simulink model "Controller_torque_cbf"  (R2026b)
settings: Solver=ode4  StopTime=Inf  FixedStep=1e-3
values from neighbouring files (symbols this model uses):
  Dn = 20 * ones(7,1)    [init_torque_cbf.m]
  H_0_cy = H_0_pr * H_pr_cy    [init_torque_cbf.m]
  H_home = getTransform(Franka_robot, q_home, 'panda_link8', 'panda_link0')    [init_torque_cbf.m]
  Kn = 0 * ones(7,1)    [init_torque_cbf.m]
  q_home = q_init    [init_torque_cbf.m]
  q_init = [0 0  0  -(2/4)*pi  0  pi/2  -pi/4]'    [init_torque_cbf.m]
undefined symbols (not defined in the file or in its folder): cbf_torque_params, DiscIntNeverNeededParam, Fext_mag, T_final, X, Y, Z
libraries: sm_lib x162, nesl_utility x44, matrix_library x3, Robotics_lib x1
(part 2 of 12)

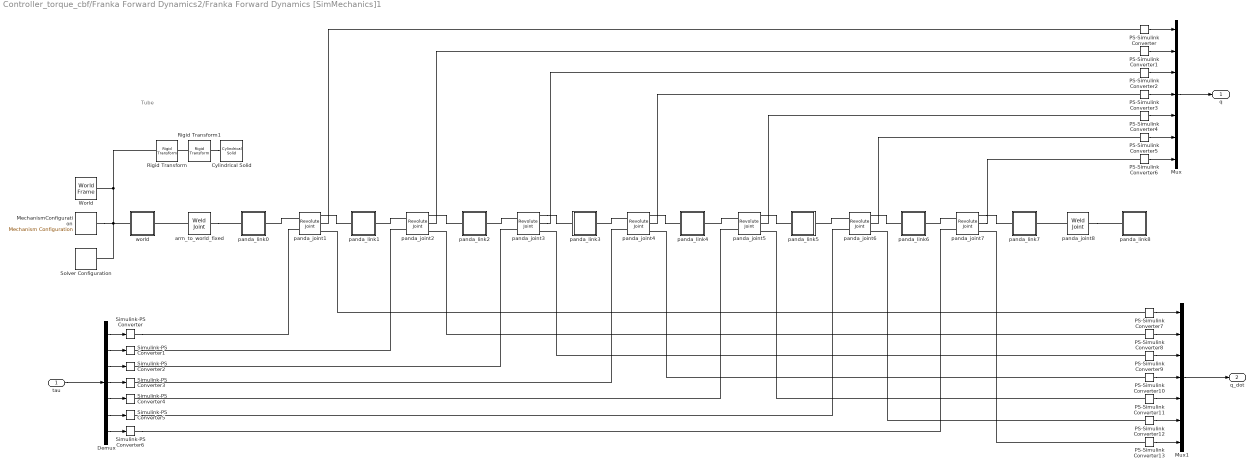
== system Controller_torque_cbf/Franka Forward Dynamics2/Franka Forward Dynamics [SimMechanics]1 ==
  note: Tube
  tau : Inport
  Cylindrical Solid : sm_lib/Body Elements/Cylindrical Solid  CylinderRadius=0.13  CylinderRadiusUnits=m  CylinderLength=0.446  CylinderLengthUnits=m  ExportEntireGeometry=off  InertiaType=CalculateFromGeometry  BasedOnType=Density  Density=1000  DensityUnits=kg/m^3  Mass=1  MassUnits=kg  CenterOfMass=[0 0 0]  CenterOfMassUnits=m  MomentsOfInertia=[1 1 1]  MomentsOfInertiaUnits=kg*m^2  ProductsOfInertia=[0 0 0]  ProductsOfInertiaUnits=kg*m^2  GraphicType=FromGeometry  MarkerShape=Sphere  MarkerSize=10  GraphicVisPropType=SimpleVisualProperties  GraphicDiffuseColor=[1.0 0.0 1.0]  GraphicOpacity=1.0  GraphicSpecularColor=[0.5 0.5 0.5 1.0]  GraphicAmbientColor=[0.15 0.15 0.15 1.0]  GraphicEmissiveColor=[0.0 0.0 0.0 1.0]  GraphicShininess=75  DoExposeReferenceFrame=on  SerializedFrames=<Frames/>
  Demux : Demux  Outputs=7
  MechanismConfiguration : sm_lib/Utilities/Mechanism Configuration  UniformGravity=Constant  GravityVector=Franka_robot.Gravity  GravityVectorUnits=m/s^2  LinearizationDelta=0.001  JointModeTransitionNonlinearIterations=2
  Mux : Mux  Inputs=7
  Mux1 : Mux  Inputs=7
  PS-Simulink Converter{,1..13} (14 alike) : nesl_utility/PS-Simulink Converter  PhysicalDomain=network_engine_domain  SubClassName=ps_output  LeftPortType=input  RightPortType=output  PseudoPeriodic=off  Frequencies=[]  VectorFormat=inherit  Unit=inherit  AffineConversion=off
  Rigid Transform : sm_lib/Frames and Transforms/Rigid Transform  RotationMethod=RotationMatrix  FollAlignAxisA=+X  BaseAlignAxisA=+Y  FollAlignAxisB=+Y  BaseAlignAxisB=+Z  RotationStandardAxis=+Z  RotationAngle=0.0  RotationAngleUnits=deg  RotationArbitraryAxis=[0 0 1]  RotationSequenceAxes=FollowerAxes  RotationSequence=XYX  RotationSequenceAngles=[0 0 0]  RotationSequenceAnglesUnits=deg  RotationMatrix=H_0_cy(1:3,1:3)  Quaternion=[1 0 0 0]  TranslationMethod=Cartesian  TranslationCartesianOffset=H_0_cy(1:3,4)  TranslationCartesianOffsetUnits=m  TranslationStandardAxis=+Z  TranslationStandardOffset=0  TranslationStandardOffsetUnits=m  TranslationROffset=0  TranslationROffsetUnits=m  TranslationThetaOffset=0  TranslationThetaOffsetUnits=deg  TranslationZOffset=0  TranslationZOffsetUnits=m
  Rigid Transform1 : sm_lib/Frames and Transforms/Rigid Transform  RotationMethod=RotationMatrix  FollAlignAxisA=+X  BaseAlignAxisA=+Y  FollAlignAxisB=+Y  BaseAlignAxisB=+Z  RotationStandardAxis=+Z  RotationAngle=0.0  RotationAngleUnits=deg  RotationArbitraryAxis=[0 0 1]  RotationSequenceAxes=FollowerAxes  RotationSequence=XYX  RotationSequenceAngles=[0 0 0]  RotationSequenceAnglesUnits=deg  RotationMatrix=[0,0,1; 0,1,0; -1,0,0]  Quaternion=[1 0 0 0]  TranslationMethod=None  TranslationCartesianOffset=zeros()  TranslationCartesianOffsetUnits=m  TranslationStandardAxis=+Z  TranslationStandardOffset=0  TranslationStandardOffsetUnits=m  TranslationROffset=0  TranslationROffsetUnits=m  TranslationThetaOffset=0  TranslationThetaOffsetUnits=deg  TranslationZOffset=0  TranslationZOffsetUnits=m
  Simulink-PS Converter{,1..6} (7 alike) : nesl_utility/Simulink-PS Converter  PhysicalDomain=network_engine_domain  SubClassName=ps_input  LeftPortType=input  RightPortType=output  PseudoPeriodic=off  Frequencies=[]  NoiseDistribution=none  NoiseParameters=[]  Unit=1  AffineConversion=off  FilteringAndDerivatives=provide  SimscapeFilterOrder=1  InputFilterTimeConstant=0.001  UdotUserProvided=0
  Solver Configuration : nesl_utility/Solver Configuration  PhysicalDomain=network_engine_domain  SubClassName=solver  LeftPortType=input  RightPortType=generic  Tones=[]  Harmonics=[]  SimulateNoise=off  Profile=off  UseLocalSampling=off  EnableSwitchedLinearOptims=on  FrequencyDomain=off  UseCCode=off  RelTol=0.001  AbsTol=0.001  MinStep=1e-09  ToWorkspace=off  RevertToSquareIcSolve=off  NumHomotopyIterations=100  PhasorMode=off  PhasorModeNumHarmonics=1  ConsistencySolver=NEWTON_XTOL_AFTER_FTOL  CanonicalOrdering=UNORDERED  OptimizeIntermediates=UNOPTIMIZED  MulticoreSolverChoice=BACKWARD_EULER  IndexReductionMethod=DerivativeReplacement  DoDC=off  ResidualTolerance=1e-09  ConsistencyTolSource=GLOBAL  ConsistencyAbsTol=0.001  ConsistencyRelTol=0.001  ConsistencyTolFactor=0.001  UseLocalSolver=off  LocalSolverChoice=NE_BACKWARD_EULER_ADVANCER  ResolveIndetEquations=on  FunctionEvalNumThread=1  LocalSolverSampleTime=0.001  DoFixedCost=off  MaxNonlinIter=3  MaxModeIter=2  ComputeImpulses=off  ImpulseIterations=2  LinearAlgebra=auto  LinearAlgebraNumThread=0  EquationFormulation=NE_TIME_EF  DelaysMemoryBudget=1024  AutomaticFiltering=on  FilteringTimeConstant=0.001  PartitionStorageMethod=AS_NEEDED  PartitionMemoryBudget=1024  PartitionMethod=BALANCED  MultibodyUseLocalSolver=off  MultibodyLocalSolverChoice=ODE1  MultibodyLocalSolverSampleTime=0.001
  World : sm_lib/Frames and Transforms/World Frame
  arm_to_world_fixed : sm_lib/Joints/Weld Joint  JointMode=Normal  CompositeWrenchDir=FollowerOnBase  CompositeWrenchFrame=BaseFrame  SenseConstraintForce=off  SenseConstraintTorque=off  SenseTotalForce=off  SenseTotalTorque=off
  panda_joint1 : sm_lib/Joints/Revolute Joint  JointMode=Normal  CompositeWrenchDir=FollowerOnBase  CompositeWrenchFrame=BaseFrame  SenseConstraintForce=off  SenseConstraintTorque=off  SenseTotalForce=off  SenseTotalTorque=off  PositionTargetSpecify=on  PositionTargetPriority=High  PositionTargetValue=q_init(1)  PositionTargetValueUnits=rad  VelocityTargetSpecify=off  VelocityTargetPriority=High  VelocityTargetValue=0  VelocityTargetValueUnits=deg/s  EquilibriumPosition=0  EquilibriumPositionUnits=deg  SpringStiffness=0  SpringStiffnessUnits=N*m/deg  DampingCoefficient=0  DampingCoefficientUnits=kg*m^2/(rad*s)  LowerLimitSpecify=on  LowerLimitBound=-2.8973  LowerLimitBoundUnits=rad  LowerLimitStiffness=1e4  LowerLimitStiffnessUnits=N*m/deg  LowerLimitDamping=10  LowerLimitDampingUnits=N*m/(deg/s)  LowerLimitTransitionRegionWidth=0.1  LowerLimitTransitionRegionWidthUnits=deg  UpperLimitSpecify=on  UpperLimitBound=2.8973  UpperLimitBoundUnits=rad  UpperLimitStiffness=1e4  UpperLimitStiffnessUnits=N*m/deg  UpperLimitDamping=10  UpperLimitDampingUnits=N*m/(deg/s)  UpperLimitTransitionRegionWidth=0.1  UpperLimitTransitionRegionWidthUnits=deg  TorqueActuationMode=InputTorque  MotionActuationMode=ComputedMotion  SensePosition=on  SenseVelocity=on  SenseAcceleration=off  SenseTorqueForce=off  SenseLowerLimitTorqueForce=off  SenseUpperLimitTorqueForce=off
  panda_joint2 : sm_lib/Joints/Revolute Joint  JointMode=Normal  CompositeWrenchDir=FollowerOnBase  CompositeWrenchFrame=BaseFrame  SenseConstraintForce=off  SenseConstraintTorque=off  SenseTotalForce=off  SenseTotalTorque=off  PositionTargetSpecify=on  PositionTargetPriority=High  PositionTargetValue=q_init(2)  PositionTargetValueUnits=rad  VelocityTargetSpecify=off  VelocityTargetPriority=High  VelocityTargetValue=0  VelocityTargetValueUnits=deg/s  EquilibriumPosition=0  EquilibriumPositionUnits=deg  SpringStiffness=0  SpringStiffnessUnits=N*m/deg  DampingCoefficient=0  DampingCoefficientUnits=kg*m^2/(rad*s)  LowerLimitSpecify=on  LowerLimitBound=-1.7628  LowerLimitBoundUnits=rad  LowerLimitStiffness=1e4  LowerLimitStiffnessUnits=N*m/deg  LowerLimitDamping=10  LowerLimitDampingUnits=N*m/(deg/s)  LowerLimitTransitionRegionWidth=0.1  LowerLimitTransitionRegionWidthUnits=deg  UpperLimitSpecify=on  UpperLimitBound=1.7628  UpperLimitBoundUnits=rad  UpperLimitStiffness=1e4  UpperLimitStiffnessUnits=N*m/deg  UpperLimitDamping=10  UpperLimitDampingUnits=N*m/(deg/s)  UpperLimitTransitionRegionWidth=0.1  UpperLimitTransitionRegionWidthUnits=deg  TorqueActuationMode=InputTorque  MotionActuationMode=ComputedMotion  SensePosition=on  SenseVelocity=on  SenseAcceleration=off  SenseTorqueForce=off  SenseLowerLimitTorqueForce=off  SenseUpperLimitTorqueForce=off
  panda_joint3 : sm_lib/Joints/Revolute Joint  JointMode=Normal  CompositeWrenchDir=FollowerOnBase  CompositeWrenchFrame=BaseFrame  SenseConstraintForce=off  SenseConstraintTorque=off  SenseTotalForce=off  SenseTotalTorque=off  PositionTargetSpecify=on  PositionTargetPriority=High  PositionTargetValue=q_init(3)  PositionTargetValueUnits=rad  VelocityTargetSpecify=off  VelocityTargetPriority=High  VelocityTargetValue=0  VelocityTargetValueUnits=deg/s  EquilibriumPosition=0  EquilibriumPositionUnits=deg  SpringStiffness=0  SpringStiffnessUnits=N*m/deg  DampingCoefficient=0  DampingCoefficientUnits=kg*m^2/(rad*s)  LowerLimitSpecify=on  LowerLimitBound=-2.8973  LowerLimitBoundUnits=rad  LowerLimitStiffness=1e4  LowerLimitStiffnessUnits=N*m/deg  LowerLimitDamping=10  LowerLimitDampingUnits=N*m/(deg/s)  LowerLimitTransitionRegionWidth=0.1  LowerLimitTransitionRegionWidthUnits=deg  UpperLimitSpecify=on  UpperLimitBound=2.8973  UpperLimitBoundUnits=rad  UpperLimitStiffness=1e4  UpperLimitStiffnessUnits=N*m/deg  UpperLimitDamping=10  UpperLimitDampingUnits=N*m/(deg/s)  UpperLimitTransitionRegionWidth=0.1  UpperLimitTransitionRegionWidthUnits=deg  TorqueActuationMode=InputTorque  MotionActuationMode=ComputedMotion  SensePosition=on  SenseVelocity=on  SenseAcceleration=off  SenseTorqueForce=off  SenseLowerLimitTorqueForce=off  SenseUpperLimitTorqueForce=off
  panda_joint4 : sm_lib/Joints/Revolute Joint  JointMode=Normal  CompositeWrenchDir=FollowerOnBase  CompositeWrenchFrame=BaseFrame  SenseConstraintForce=off  SenseConstraintTorque=off  SenseTotalForce=off  SenseTotalTorque=off  PositionTargetSpecify=on  PositionTargetPriority=High  PositionTargetValue=q_init(4)  PositionTargetValueUnits=rad  VelocityTargetSpecify=off  VelocityTargetPriority=High  VelocityTargetValue=0  VelocityTargetValueUnits=deg/s  EquilibriumPosition=0  EquilibriumPositionUnits=deg  SpringStiffness=0  SpringStiffnessUnits=N*m/deg  DampingCoefficient=0  DampingCoefficientUnits=kg*m^2/(rad*s)  LowerLimitSpecify=on  LowerLimitBound=-3.0718  LowerLimitBoundUnits=rad  LowerLimitStiffness=1e4  LowerLimitStiffnessUnits=N*m/deg  LowerLimitDamping=10  LowerLimitDampingUnits=N*m/(deg/s)  LowerLimitTransitionRegionWidth=0.1  LowerLimitTransitionRegionWidthUnits=deg  UpperLimitSpecify=on  UpperLimitBound=-0.0698  UpperLimitBoundUnits=rad  UpperLimitStiffness=1e4  UpperLimitStiffnessUnits=N*m/deg  UpperLimitDamping=10  UpperLimitDampingUnits=N*m/(deg/s)  UpperLimitTransitionRegionWidth=0.1  UpperLimitTransitionRegionWidthUnits=deg  TorqueActuationMode=InputTorque  MotionActuationMode=ComputedMotion  SensePosition=on  SenseVelocity=on  SenseAcceleration=off  SenseTorqueForce=off  SenseLowerLimitTorqueForce=off  SenseUpperLimitTorqueForce=off
  panda_joint5 : sm_lib/Joints/Revolute Joint  JointMode=Normal  CompositeWrenchDir=FollowerOnBase  CompositeWrenchFrame=BaseFrame  SenseConstraintForce=off  SenseConstraintTorque=off  SenseTotalForce=off  SenseTotalTorque=off  PositionTargetSpecify=on  PositionTargetPriority=High  PositionTargetValue=q_init(5)  PositionTargetValueUnits=rad  VelocityTargetSpecify=off  VelocityTargetPriority=High  VelocityTargetValue=0  VelocityTargetValueUnits=deg/s  EquilibriumPosition=0  EquilibriumPositionUnits=deg  SpringStiffness=0  SpringStiffnessUnits=N*m/deg  DampingCoefficient=0  DampingCoefficientUnits=kg*m^2/(rad*s)  LowerLimitSpecify=on  LowerLimitBound=-2.8973  LowerLimitBoundUnits=rad  LowerLimitStiffness=1e4  LowerLimitStiffnessUnits=N*m/deg  LowerLimitDamping=10  LowerLimitDampingUnits=N*m/(deg/s)  LowerLimitTransitionRegionWidth=0.1  LowerLimitTransitionRegionWidthUnits=deg  UpperLimitSpecify=on  UpperLimitBound=2.8973  UpperLimitBoundUnits=rad  UpperLimitStiffness=1e4  UpperLimitStiffnessUnits=N*m/deg  UpperLimitDamping=10  UpperLimitDampingUnits=N*m/(deg/s)  UpperLimitTransitionRegionWidth=0.1  UpperLimitTransitionRegionWidthUnits=deg  TorqueActuationMode=InputTorque  MotionActuationMode=ComputedMotion  SensePosition=on  SenseVelocity=on  SenseAcceleration=off  SenseTorqueForce=off  SenseLowerLimitTorqueForce=off  SenseUpperLimitTorqueForce=off
  panda_joint6 : sm_lib/Joints/Revolute Joint  JointMode=Normal  CompositeWrenchDir=FollowerOnBase  CompositeWrenchFrame=BaseFrame  SenseConstraintForce=off  SenseConstraintTorque=off  SenseTotalForce=off  SenseTotalTorque=off  PositionTargetSpecify=on  PositionTargetPriority=High  PositionTargetValue=q_init(6)  PositionTargetValueUnits=rad  VelocityTargetSpecify=off  VelocityTargetPriority=High  VelocityTargetValue=0  VelocityTargetValueUnits=deg/s  EquilibriumPosition=0  EquilibriumPositionUnits=deg  SpringStiffness=0  SpringStiffnessUnits=N*m/deg  DampingCoefficient=0  DampingCoefficientUnits=kg*m^2/(rad*s)  LowerLimitSpecify=on  LowerLimitBound=-0.0175  LowerLimitBoundUnits=rad  LowerLimitStiffness=1e4  LowerLimitStiffnessUnits=N*m/deg  LowerLimitDamping=10  LowerLimitDampingUnits=N*m/(deg/s)  LowerLimitTransitionRegionWidth=0.1  LowerLimitTransitionRegionWidthUnits=deg  UpperLimitSpecify=on  UpperLimitBound=3.7525  UpperLimitBoundUnits=rad  UpperLimitStiffness=1e4  UpperLimitStiffnessUnits=N*m/deg  UpperLimitDamping=10  UpperLimitDampingUnits=N*m/(deg/s)  UpperLimitTransitionRegionWidth=0.1  UpperLimitTransitionRegionWidthUnits=deg  TorqueActuationMode=InputTorque  MotionActuationMode=ComputedMotion  SensePosition=on  SenseVelocity=on  SenseAcceleration=off  SenseTorqueForce=off  SenseLowerLimitTorqueForce=off  SenseUpperLimitTorqueForce=off
  panda_joint7 : sm_lib/Joints/Revolute Joint  JointMode=Normal  CompositeWrenchDir=FollowerOnBase  CompositeWrenchFrame=BaseFrame  SenseConstraintForce=off  SenseConstraintTorque=off  SenseTotalForce=off  SenseTotalTorque=off  PositionTargetSpecify=on  PositionTargetPriority=High  PositionTargetValue=q_init(7)  PositionTargetValueUnits=rad  VelocityTargetSpecify=off  VelocityTargetPriority=High  VelocityTargetValue=0  VelocityTargetValueUnits=deg/s  EquilibriumPosition=0  EquilibriumPositionUnits=deg  SpringStiffness=0  SpringStiffnessUnits=N*m/deg  DampingCoefficient=0  DampingCoefficientUnits=kg*m^2/(rad*s)  LowerLimitSpecify=on  LowerLimitBound=-2.8973  LowerLimitBoundUnits=rad  LowerLimitStiffness=1e4  LowerLimitStiffnessUnits=N*m/deg  LowerLimitDamping=10  LowerLimitDampingUnits=N*m/(deg/s)  LowerLimitTransitionRegionWidth=0.1  LowerLimitTransitionRegionWidthUnits=deg  UpperLimitSpecify=on  UpperLimitBound=2.8973  UpperLimitBoundUnits=rad  UpperLimitStiffness=1e4  UpperLimitStiffnessUnits=N*m/deg  UpperLimitDamping=10  UpperLimitDampingUnits=N*m/(deg/s)  UpperLimitTransitionRegionWidth=0.1  UpperLimitTransitionRegionWidthUnits=deg  TorqueActuationMode=InputTorque  MotionActuationMode=ComputedMotion  SensePosition=on  SenseVelocity=on  SenseAcceleration=off  SenseTorqueForce=off  SenseLowerLimitTorqueForce=off  SenseUpperLimitTorqueForce=off
  panda_joint8 : sm_lib/Joints/Weld Joint  JointMode=Normal  CompositeWrenchDir=FollowerOnBase  CompositeWrenchFrame=BaseFrame  SenseConstraintForce=off  SenseConstraintTorque=off  SenseTotalForce=off  SenseTotalTorque=off
  panda_link0 : Subsystem
  panda_link1 : Subsystem
  panda_link2 : Subsystem
  panda_link3 : Subsystem
  panda_link4 : Subsystem
  panda_link5 : Subsystem
  panda_link6 : Subsystem
  panda_link7 : Subsystem
  panda_link8 : Subsystem
  world : Subsystem
  q : Outport
  q_dot : Outport  Port=2
  wires:
  Demux/6 -> Simulink-PS Converter5/1
  PS-Simulink Converter4/1 -> Mux/5
  PS-Simulink Converter8/1 -> Mux1/2
  tau/1 -> Demux/1
  PS-Simulink Converter11/1 -> Mux1/5
  PS-Simulink Converter2/1 -> Mux/3
  PS-Simulink Converter5/1 -> Mux/6
  Demux/5 -> Simulink-PS Converter4/1
  PS-Simulink Converter7/1 -> Mux1/1
  PS-Simulink Converter3/1 -> Mux/4
  Mux1/1 -> q_dot/1
  Demux/7 -> Simulink-PS Converter6/1
  Demux/4 -> Simulink-PS Converter3/1
  Demux/1 -> Simulink-PS Converter/1
  PS-Simulink Converter10/1 -> Mux1/4
  PS-Simulink Converter/1 -> Mux/1
  PS-Simulink Converter9/1 -> Mux1/3
  Demux/3 -> Simulink-PS Converter2/1
  PS-Simulink Converter6/1 -> Mux/7
  PS-Simulink Converter13/1 -> Mux1/7
  PS-Simulink Converter12/1 -> Mux1/6
  Demux/2 -> Simulink-PS Converter1/1
  PS-Simulink Converter1/1 -> Mux/2
  Mux/1 -> q/1
  connections:
  PS-Simulink Converter8/LConn1 -- panda_joint2/RConn3
  panda_joint8/RConn1 -- panda_link8/LConn1
  panda_joint2/RConn1 -- panda_link2/LConn1
  PS-Simulink Converter11/LConn1 -- panda_joint5/RConn3
  Simulink-PS Converter5/RConn1 -- panda_joint6/LConn2
  Solver Configuration/RConn1 -- world/LConn1 -- MechanismConfiguration/RConn1 -- Rigid Transform/LConn1 -- World/RConn1
  PS-Simulink Converter10/LConn1 -- panda_joint4/RConn3
  panda_joint2/LConn1 -- panda_link1/RConn1
  panda_joint7/RConn2 -- PS-Simulink Converter6/LConn1
  arm_to_world_fixed/RConn1 -- panda_link0/LConn1
  panda_joint6/RConn2 -- PS-Simulink Converter5/LConn1
  PS-Simulink Converter9/LConn1 -- panda_joint3/RConn3
  panda_joint4/RConn1 -- panda_link4/LConn1
  panda_joint7/RConn1 -- panda_link7/LConn1
  panda_joint2/RConn2 -- PS-Simulink Converter1/LConn1
  panda_joint4/RConn2 -- PS-Simulink Converter3/LConn1
  panda_joint4/LConn1 -- panda_link3/RConn1
  PS-Simulink Converter12/LConn1 -- panda_joint6/RConn3
  panda_joint3/RConn2 -- PS-Simulink Converter2/LConn1
  Simulink-PS Converter/RConn1 -- panda_joint1/LConn2
  panda_joint3/LConn1 -- panda_link2/RConn1
  panda_joint1/RConn1 -- panda_link1/LConn1
  panda_joint3/RConn1 -- panda_link3/LConn1
  PS-Simulink Converter7/LConn1 -- panda_joint1/RConn3
  panda_joint1/RConn2 -- PS-Simulink Converter/LConn1
  panda_joint1/LConn1 -- panda_link0/RConn1
  panda_joint5/RConn1 -- panda_link5/LConn1
  panda_joint6/RConn1 -- panda_link6/LConn1
  Simulink-PS Converter1/RConn1 -- panda_joint2/LConn2
  Simulink-PS Converter6/RConn1 -- panda_joint7/LConn2
  arm_to_world_fixed/LConn1 -- world/RConn1
  panda_joint7/LConn1 -- panda_link6/RConn1
  panda_joint5/LConn1 -- panda_link4/RConn1
  panda_joint8/LConn1 -- panda_link7/RConn1
  PS-Simulink Converter13/LConn1 -- panda_joint7/RConn3
  Simulink-PS Converter4/RConn1 -- panda_joint5/LConn2
  Simulink-PS Converter2/RConn1 -- panda_joint3/LConn2
  panda_joint6/LConn1 -- panda_link5/RConn1
  Simulink-PS Converter3/RConn1 -- panda_joint4/LConn2
  panda_joint5/RConn2 -- PS-Simulink Converter4/LConn1
  Rigid Transform1/RConn1 -- Cylindrical Solid/RConn1
  Rigid Transform1/LConn1 -- Rigid Transform/RConn1

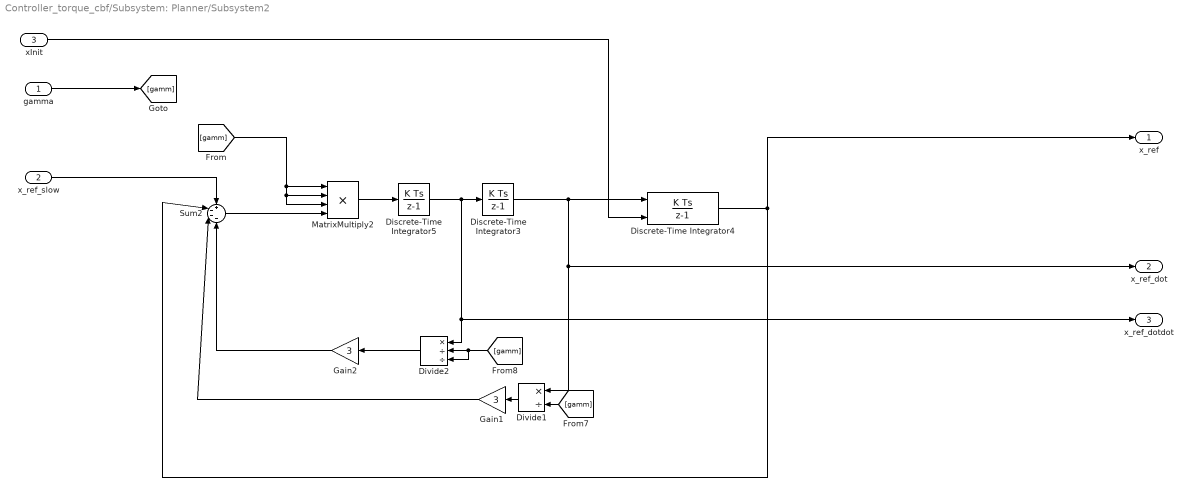
== system Controller_torque_cbf/Subsystem: Planner/Subsystem2 ==
  gamma : Inport
  x_ref_slow : Inport  Port=2
  xInit : Inport  Port=3
  Discrete-Time Integrator3 : DiscreteIntegrator  SampleTime=-1  ICPrevOutput=DiscIntNeverNeededParam  ICPrevScaledInput=DiscIntNeverNeededParam
  Discrete-Time Integrator4 : DiscreteIntegrator  InitialConditionSource=external  SampleTime=-1  ICPrevOutput=DiscIntNeverNeededParam  ICPrevScaledInput=DiscIntNeverNeededParam
  Discrete-Time Integrator5 : DiscreteIntegrator  SampleTime=-1  ICPrevOutput=DiscIntNeverNeededParam  ICPrevScaledInput=DiscIntNeverNeededParam
  Divide1 : Product  Inputs=*/
  Divide2 : Product  Inputs=*//
  Gain1 : Gain  Gain=3
  Gain2 : Gain  Gain=3
  MatrixMultiply2 : Product  Inputs=4
  Sum2 : Sum  Inputs=+---
  x_ref : Outport
  x_ref_dot : Outport  Port=2
  x_ref_dotdot : Outport  Port=3
  wires:
  Divide2/1 -> Gain2/1
  gamma/1 -> [gamm]
  [gamm] -> Divide2/3, Divide2/2
  Divide1/1 -> Gain1/1
  Sum2/1 -> MatrixMultiply2/4
  Gain2/1 -> Sum2/4
  [gamm] -> Divide1/2
  xInit/1 -> Discrete-Time Integrator4/2
  Discrete-Time Integrator3/1 -> x_ref_dot/1, Divide1/1, Discrete-Time Integrator4/1
  Gain1/1 -> Sum2/3
  Discrete-Time Integrator5/1 -> Discrete-Time Integrator3/1, x_ref_dotdot/1, Divide2/1
  Discrete-Time Integrator4/1 -> x_ref/1, Sum2/2
  MatrixMultiply2/1 -> Discrete-Time Integrator5/1
  x_ref_slow/1 -> Sum2/1
  [gamm] -> MatrixMultiply2/3, MatrixMultiply2/2, MatrixMultiply2/1

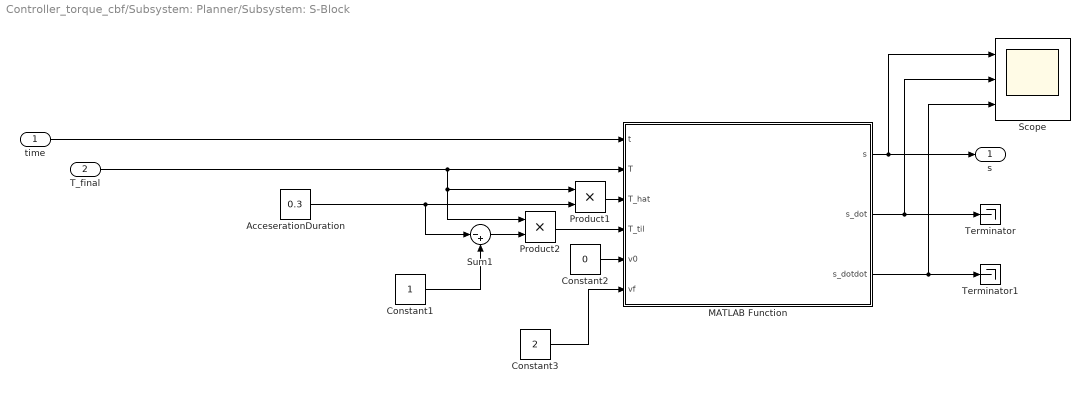
== system Controller_torque_cbf/Subsystem: Planner/Subsystem: S-Block ==
  time : Inport
  T_final : Inport  Port=2
  AcceserationDuration : Constant  Value=0.3
  Constant1 : Constant
  Constant2 : Constant  Value=0
  Constant3 : Constant  Value=2
  MATLAB Function : MATLAB Function  TreatAsAtomicUnit=on
  Product1 : Product
  Product2 : Product
  Scope : Scope  NumInputPorts=3
      settings: ActiveDisplayYMinimum=-0.125  ActiveDisplayYMaximum=1.125  DataLoggingVariableName=ScopeData2
  Sum1 : Sum  Inputs=|-+
  Terminator : Terminator
  Terminator1 : Terminator
  s : Outport
  wires:
  Constant2/1 -> MATLAB Function/5(v0)
  T_final/1 -> Product2/1, Product1/1, MATLAB Function/2(T)
  AcceserationDuration/1 -> Sum1/1, Product1/2
  Sum1/1 -> Product2/2
  Product2/1 -> MATLAB Function/4(T_til)
  Product1/1 -> MATLAB Function/3(T_hat)
  Constant1/1 -> Sum1/2
  MATLAB Function/1(s) -> Scope/1, s/1
  time/1 -> MATLAB Function/1(t)
  MATLAB Function/2(s_dot) -> Scope/2, Terminator/1
  MATLAB Function/3(s_dotdot) -> Scope/3, Terminator1/1
  Constant3/1 -> MATLAB Function/6(vf)

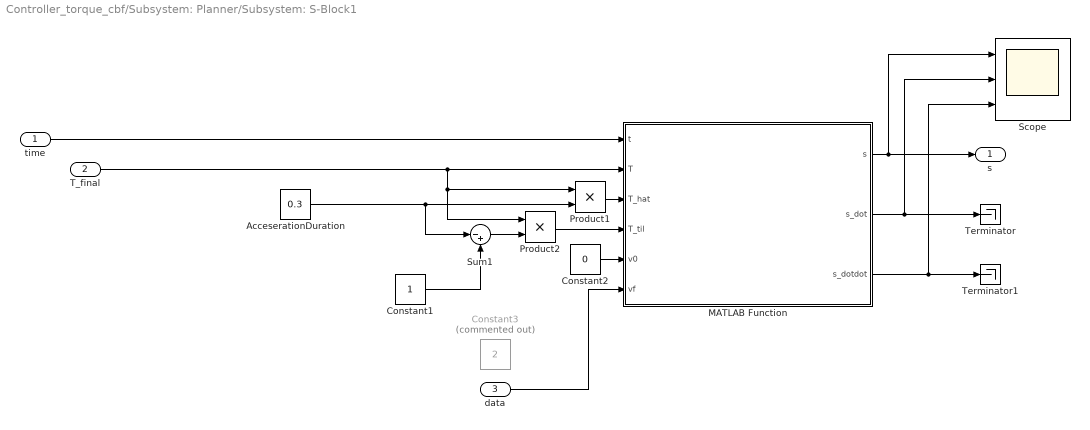
== system Controller_torque_cbf/Subsystem: Planner/Subsystem: S-Block1 ==
  time : Inport
  T_final : Inport  Port=2
  data : Inport  Port=3
  AcceserationDuration : Constant  Value=0.3
  Constant1 : Constant
  Constant2 : Constant  Value=0
  Constant3 : Constant  Commented=on  Value=2
  MATLAB Function : MATLAB Function  TreatAsAtomicUnit=on
  Product1 : Product
  Product2 : Product
  Scope : Scope  NumInputPorts=3
      settings: ActiveDisplayYMinimum=-0.125  ActiveDisplayYMaximum=1.125  DataLoggingVariableName=ScopeData2
  Sum1 : Sum  Inputs=|-+
  Terminator : Terminator
  Terminator1 : Terminator
  s : Outport
  wires:
  Constant2/1 -> MATLAB Function/5(v0)
  T_final/1 -> Product2/1, Product1/1, MATLAB Function/2(T)
  AcceserationDuration/1 -> Sum1/1, Product1/2
  Sum1/1 -> Product2/2
  Product2/1 -> MATLAB Function/4(T_til)
  Product1/1 -> MATLAB Function/3(T_hat)
  Constant1/1 -> Sum1/2
  MATLAB Function/1(s) -> Scope/1, s/1
  time/1 -> MATLAB Function/1(t)
  MATLAB Function/2(s_dot) -> Scope/2, Terminator/1
  MATLAB Function/3(s_dotdot) -> Scope/3, Terminator1/1
  data/1 -> MATLAB Function/6(vf)

== system Controller_torque_cbf/task space controller/CBF_Telemetry_Visualizer ==
  telem : Inport
  Demux : Demux  Outputs=8
  Mux_ActSlack : Mux  Inputs=2
  Mux_PhaseSpace : Mux  Inputs=2
  Scope_Activity_and_Slack : Scope
  Scope_Barrier_B : Scope
  Scope_Braking_Force_fn : Scope
  Scope_Distance_zeta : Scope
  Scope_QP_Cost : Scope
  Scope_Velocity_vs_Envelope : Scope
  wires:
  telem/1 -> Demux/1
  Demux/2 -> Scope_Distance_zeta/1
  Demux/3 -> Mux_PhaseSpace/1
  Demux/4 -> Mux_PhaseSpace/2
  Mux_PhaseSpace/1 -> Scope_Velocity_vs_Envelope/1
  Demux/5 -> Scope_Barrier_B/1
  Demux/6 -> Scope_Braking_Force_fn/1
  Demux/1 -> Mux_ActSlack/1
  Demux/7 -> Mux_ActSlack/2
  Mux_ActSlack/1 -> Scope_Activity_and_Slack/1
  Demux/8 -> Scope_QP_Cost/1

== system Controller_torque_cbf/task space controller/Damping Desing Selection ==
  Lambda_mat : Inport
  Kd : Inport  Port=2
  Damping Matrix Design : MATLAB Function  TreatAsAtomicUnit=on
  MATLAB Function2 : MATLAB Function  TreatAsAtomicUnit=on
  Memory : Memory  InitialCondition=eye(6)  InheritSampleTime=on
  K_ref : Outport
  D_ref : Outport  Port=2
  wires:
  Memory/1 -> Damping Matrix Design/3(Q_old)
  Damping Matrix Design/4(Qret) -> Memory/1
  Lambda_mat/1 -> Damping Matrix Design/1(M)
  Damping Matrix Design/3(xi_vec) -> MATLAB Function2/3(xi_vec)
  MATLAB Function2/1(K_d) -> K_ref/1
  MATLAB Function2/2(D_d) -> D_ref/1
  Damping Matrix Design/2(v_vec) -> MATLAB Function2/2(v_vec)
  Damping Matrix Design/1(LQ) -> MATLAB Function2/1(LQ)
  Kd/1 -> Damping Matrix Design/2(K)

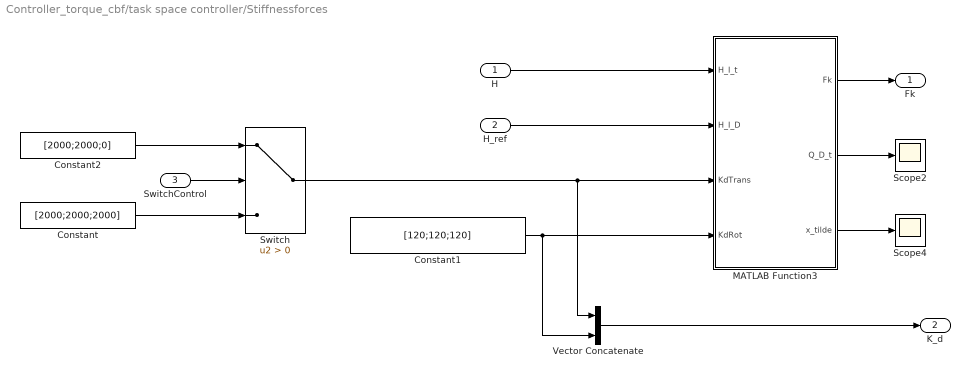
== system Controller_torque_cbf/task space controller/Stiffnessforces ==
  H : Inport
  H_ref : Inport  Port=2
  SwitchControl : Inport  Port=3
  Constant : Constant  Value=[2000;2000;2000]
  Constant1 : Constant  Value=[120;120;120]
  Constant2 : Constant  Value=[2000;2000;0]
  MATLAB Function3 : MATLAB Function  TreatAsAtomicUnit=on
  Scope2 : Scope
      settings: ActiveDisplayYMinimum=-0.1267  ActiveDisplayYMaximum=1.12519  DataLoggingVariableName=ScopeData5
  Scope4 : Scope
      settings: DataLoggingVariableName=ScopeData6
  Switch : Switch  Criteria=u2 > Threshold  SaturateOnIntegerOverflow=off  InputSameDT=off
  Vector Concatenate : Concatenate
  Fk : Outport
  K_d : Outport  Port=2
  wires:
  Switch/1 -> Vector Concatenate/1, MATLAB Function3/3(KdTrans)
  Constant1/1 -> Vector Concatenate/2, MATLAB Function3/4(KdRot)
  H_ref/1 -> MATLAB Function3/2(H_I_D)
  H/1 -> MATLAB Function3/1(H_I_t)
  MATLAB Function3/2(Q_D_t) -> Scope2/1
  MATLAB Function3/3(x_tilde) -> Scope4/1
  MATLAB Function3/1(Fk) -> Fk/1
  Vector Concatenate/1 -> K_d/1
  SwitchControl/1 -> Switch/2
  Constant2/1 -> Switch/1
  Constant/1 -> Switch/3

== system Controller_torque_cbf/task space controller/Subsystem2 ==
  u : Inport
  Constant : Constant  Value=100
  Discrete-Time Integrator : DiscreteIntegrator  SampleTime=-1  ICPrevOutput=DiscIntNeverNeededParam  ICPrevScaledInput=DiscIntNeverNeededParam
  MatrixMultiply : Product
  Sum : Sum  Inputs=|+-
  x : Outport
  wires:
  u/1 -> Sum/1
  Sum/1 -> MatrixMultiply/2
  Constant/1 -> MatrixMultiply/1
  MatrixMultiply/1 -> Discrete-Time Integrator/1
  Discrete-Time Integrator/1 -> Sum/2, x/1

== system Controller_torque_cbf/task space controller/Subsystem4 ==
  q_dot : Inport
  Jg : Inport  Port=2
  V_body_ref : Inport  Port=3
  Htm : Inport  Port=4
  H_ref : Inport  Port=5
  MATLAB Function : MATLAB Function  TreatAsAtomicUnit=on
  V_tilde : Outport
  wires:
  MATLAB Function/1(V_tilde) -> V_tilde/1
  Jg/1 -> MATLAB Function/2(Jg)
  q_dot/1 -> MATLAB Function/1(q_dot)
  Htm/1 -> MATLAB Function/4(H_I_t)
  H_ref/1 -> MATLAB Function/5(H_I_D)
  V_body_ref/1 -> MATLAB Function/3(V_body_ref)

== system Controller_torque_cbf/Franka Forward Dynamics2/Franka Forward Dynamics [SimMechanics]/panda_link0 ==
  Inertia : sm_lib/Body Elements/Inertia  InertiaType=Custom  Mass=0.629769  MassUnits=kg  CenterOfMass=[0, 0, 0]  CenterOfMassUnits=m  MomentsOfInertia=[0.00315, 0.003880000000000001, 0.004285]  MomentsOfInertiaUnits=kg*m^2  ProductsOfInertia=[8.229900000000001e-06, 0.00015, 8.290399999999999e-07]  ProductsOfInertiaUnits=kg*m^2  GraphicType=None  MarkerShape=Inertia  MarkerSize=20  GraphicVisPropType=SimpleVisualProperties  GraphicDiffuseColor=[0.5 0.5 0.5]  GraphicOpacity=1.0  GraphicSpecularColor=[0.5 0.5 0.5 1.0]  GraphicAmbientColor=[0.15 0.15 0.15 1.0]  GraphicEmissiveColor=[0.0 0.0 0.0 1.0]  GraphicShininess=75
  InertiaOriginTransform : sm_lib/Frames and Transforms/Rigid Transform  RotationMethod=RotationSequence  FollAlignAxisA=+X  BaseAlignAxisA=+Y  FollAlignAxisB=+Y  BaseAlignAxisB=+Z  RotationStandardAxis=+Z  RotationAngle=0.0  RotationAngleUnits=deg  RotationArbitraryAxis=[0 0 1]  RotationSequenceAxes=BaseAxes  RotationSequence=XYZ  RotationSequenceAngles=[0, 0, 0]  RotationSequenceAnglesUnits=rad  RotationMatrix=[1 0 0; 0 1 0; 0 0 1]  Quaternion=[1 0 0 0]  TranslationMethod=Cartesian  TranslationCartesianOffset=[-0.041018, -0.00014, 0.049974]  TranslationCartesianOffsetUnits=m  TranslationStandardAxis=+Z  TranslationStandardOffset=0  TranslationStandardOffsetUnits=m  TranslationROffset=0  TranslationROffsetUnits=m  TranslationThetaOffset=0  TranslationThetaOffsetUnits=deg  TranslationZOffset=0  TranslationZOffsetUnits=m
  ReferenceFrame : sm_lib/Frames and Transforms/Reference Frame
  Visual : sm_lib/Body Elements/File Solid  ExtGeomFileName=RobotFiles/Franka_Panda/meshes/visual/link0.stl  UnitType=Custom  ExtGeomFileUnits=mm  StepReaderType=HEX  ExportConvexHullGeometry=off  InertiaType=Custom  BasedOnType=DensityFromFile  Density=1000  DensityUnits=kg/m^3  Mass=0  MassUnits=kg  CenterOfMass=[0, 0, 0]  CenterOfMassUnits=m  MomentsOfInertia=[0, 0, 0]  MomentsOfInertiaUnits=kg*m^2  ProductsOfInertia=[0, 0, 0]  ProductsOfInertiaUnits=kg*m^2  GraphicType=FromGeometry  MarkerShape=Sphere  MarkerSize=10  GraphicVisPropType=SimpleVisualProperties  GraphicDiffuseColor=[1.0 1.0 1.0]  GraphicOpacity=1  GraphicSpecularColor=[0.5 0.5 0.5 1.0]  GraphicAmbientColor=[0.15 0.15 0.15 1.0]  GraphicEmissiveColor=[0.0 0.0 0.0 1.0]  GraphicShininess=75  DoExposeReferenceFrame=on  SerializedFrames=<Frames/>
  VisualOriginTransform : sm_lib/Frames and Transforms/Rigid Transform  RotationMethod=RotationSequence  FollAlignAxisA=+X  BaseAlignAxisA=+Y  FollAlignAxisB=+Y  BaseAlignAxisB=+Z  RotationStandardAxis=+Z  RotationAngle=0.0  RotationAngleUnits=deg  RotationArbitraryAxis=[0 0 1]  RotationSequenceAxes=BaseAxes  RotationSequence=XYZ  RotationSequenceAngles=[0, 0, 0]  RotationSequenceAnglesUnits=rad  RotationMatrix=[1 0 0; 0 1 0; 0 0 1]  Quaternion=[1 0 0 0]  TranslationMethod=Cartesian  TranslationCartesianOffset=[0, 0, 0]  TranslationCartesianOffsetUnits=m  TranslationStandardAxis=+Z  TranslationStandardOffset=0  TranslationStandardOffsetUnits=m  TranslationROffset=0  TranslationROffsetUnits=m  TranslationThetaOffset=0  TranslationThetaOffsetUnits=deg  TranslationZOffset=0  TranslationZOffsetUnits=m
  panda_joint1_AxisTransform : sm_lib/Frames and Transforms/Rigid Transform  RotationMethod=ArbitraryAxis  FollAlignAxisA=+X  BaseAlignAxisA=+Y  FollAlignAxisB=+Y  BaseAlignAxisB=+Z  RotationStandardAxis=+Z  RotationAngle=0  RotationAngleUnits=rad  RotationArbitraryAxis=[1, 0, 0]  RotationSequenceAxes=FollowerAxes  RotationSequence=XYX  RotationSequenceAngles=[0 0 0]  RotationSequenceAnglesUnits=deg  RotationMatrix=[1 0 0; 0 1 0; 0 0 1]  Quaternion=[1 0 0 0]  TranslationMethod=Cartesian  TranslationCartesianOffset=[0, 0, 0]  TranslationCartesianOffsetUnits=m  TranslationStandardAxis=+Z  TranslationStandardOffset=0  TranslationStandardOffsetUnits=m  TranslationROffset=0  TranslationROffsetUnits=m  TranslationThetaOffset=0  TranslationThetaOffsetUnits=deg  TranslationZOffset=0  TranslationZOffsetUnits=m
  panda_joint1_OriginTransform : sm_lib/Frames and Transforms/Rigid Transform  RotationMethod=RotationSequence  FollAlignAxisA=+X  BaseAlignAxisA=+Y  FollAlignAxisB=+Y  BaseAlignAxisB=+Z  RotationStandardAxis=+Z  RotationAngle=0.0  RotationAngleUnits=deg  RotationArbitraryAxis=[0 0 1]  RotationSequenceAxes=BaseAxes  RotationSequence=XYZ  RotationSequenceAngles=[0, 0, 0]  RotationSequenceAnglesUnits=rad  RotationMatrix=[1 0 0; 0 1 0; 0 0 1]  Quaternion=[1 0 0 0]  TranslationMethod=Cartesian  TranslationCartesianOffset=[0, 0, 0.333]  TranslationCartesianOffsetUnits=m  TranslationStandardAxis=+Z  TranslationStandardOffset=0  TranslationStandardOffsetUnits=m  TranslationROffset=0  TranslationROffsetUnits=m  TranslationThetaOffset=0  TranslationThetaOffsetUnits=deg  TranslationZOffset=0  TranslationZOffsetUnits=m
  F : PMIOPort  Side=Left
  F1 : PMIOPort  Port=2  Side=Right
  connections:
  Inertia/RConn1 -- InertiaOriginTransform/RConn1
  ReferenceFrame/RConn1 -- InertiaOriginTransform/LConn1 -- VisualOriginTransform/LConn1 -- panda_joint1_OriginTransform/LConn1 -- F/RConn1
  Visual/RConn1 -- VisualOriginTransform/RConn1
  panda_joint1_AxisTransform/RConn1 -- F1/RConn1
  panda_joint1_AxisTransform/LConn1 -- panda_joint1_OriginTransform/RConn1

== system Controller_torque_cbf/Franka Forward Dynamics2/Franka Forward Dynamics [SimMechanics]/panda_link1 ==
  Inertia : sm_lib/Body Elements/Inertia  InertiaType=Custom  Mass=4.970684  MassUnits=kg  CenterOfMass=[0, 0, 0]  CenterOfMassUnits=m  MomentsOfInertia=[0.7033700000000001, 0.70661, 0.009117]  MomentsOfInertiaUnits=kg*m^2  ProductsOfInertia=[0.019169, 0.006772, -0.000139]  ProductsOfInertiaUnits=kg*m^2  GraphicType=None  MarkerShape=Inertia  MarkerSize=20  GraphicVisPropType=SimpleVisualProperties  GraphicDiffuseColor=[0.5 0.5 0.5]  GraphicOpacity=1.0  GraphicSpecularColor=[0.5 0.5 0.5 1.0]  GraphicAmbientColor=[0.15 0.15 0.15 1.0]  GraphicEmissiveColor=[0.0 0.0 0.0 1.0]  GraphicShininess=75
  InertiaOriginTransform : sm_lib/Frames and Transforms/Rigid Transform  RotationMethod=RotationSequence  FollAlignAxisA=+X  BaseAlignAxisA=+Y  FollAlignAxisB=+Y  BaseAlignAxisB=+Z  RotationStandardAxis=+Z  RotationAngle=0.0  RotationAngleUnits=deg  RotationArbitraryAxis=[0 0 1]  RotationSequenceAxes=BaseAxes  RotationSequence=XYZ  RotationSequenceAngles=[0, 0, 0]  RotationSequenceAnglesUnits=rad  RotationMatrix=[1 0 0; 0 1 0; 0 0 1]  Quaternion=[1 0 0 0]  TranslationMethod=Cartesian  TranslationCartesianOffset=[0.003875, 0.002081, -0.04762]  TranslationCartesianOffsetUnits=m  TranslationStandardAxis=+Z  TranslationStandardOffset=0  TranslationStandardOffsetUnits=m  TranslationROffset=0  TranslationROffsetUnits=m  TranslationThetaOffset=0  TranslationThetaOffsetUnits=deg  TranslationZOffset=0  TranslationZOffsetUnits=m
  ReferenceFrame : sm_lib/Frames and Transforms/Reference Frame
  Visual : sm_lib/Body Elements/File Solid  ExtGeomFileName=RobotFiles/Franka_Panda/meshes/visual/link1-Mesh.stl  UnitType=Custom  ExtGeomFileUnits=mm  StepReaderType=HEX  ExportConvexHullGeometry=off  InertiaType=Custom  BasedOnType=DensityFromFile  Density=1000  DensityUnits=kg/m^3  Mass=0  MassUnits=kg  CenterOfMass=[0, 0, 0]  CenterOfMassUnits=m  MomentsOfInertia=[0, 0, 0]  MomentsOfInertiaUnits=kg*m^2  ProductsOfInertia=[0, 0, 0]  ProductsOfInertiaUnits=kg*m^2  GraphicType=FromGeometry  MarkerShape=Sphere  MarkerSize=10  GraphicVisPropType=SimpleVisualProperties  GraphicDiffuseColor=[1.0 1.0 1.0]  GraphicOpacity=1  GraphicSpecularColor=[0.5 0.5 0.5 1.0]  GraphicAmbientColor=[0.15 0.15 0.15 1.0]  GraphicEmissiveColor=[0.0 0.0 0.0 1.0]  GraphicShininess=75  DoExposeReferenceFrame=on  SerializedFrames=<Frames/>
  VisualOriginTransform : sm_lib/Frames and Transforms/Rigid Transform  RotationMethod=RotationSequence  FollAlignAxisA=+X  BaseAlignAxisA=+Y  FollAlignAxisB=+Y  BaseAlignAxisB=+Z  RotationStandardAxis=+Z  RotationAngle=0.0  RotationAngleUnits=deg  RotationArbitraryAxis=[0 0 1]  RotationSequenceAxes=BaseAxes  RotationSequence=XYZ  RotationSequenceAngles=[0, 0, 0]  RotationSequenceAnglesUnits=rad  RotationMatrix=[1 0 0; 0 1 0; 0 0 1]  Quaternion=[1 0 0 0]  TranslationMethod=Cartesian  TranslationCartesianOffset=[0, 0, 0]  TranslationCartesianOffsetUnits=m  TranslationStandardAxis=+Z  TranslationStandardOffset=0  TranslationStandardOffsetUnits=m  TranslationROffset=0  TranslationROffsetUnits=m  TranslationThetaOffset=0  TranslationThetaOffsetUnits=deg  TranslationZOffset=0  TranslationZOffsetUnits=m
  panda_joint1_AxisInvTransform : sm_lib/Frames and Transforms/Rigid Transform  RotationMethod=ArbitraryAxis  FollAlignAxisA=+X  BaseAlignAxisA=+Y  FollAlignAxisB=+Y  BaseAlignAxisB=+Z  RotationStandardAxis=+Z  RotationAngle=0  RotationAngleUnits=rad  RotationArbitraryAxis=[1, 0, 0]  RotationSequenceAxes=FollowerAxes  RotationSequence=XYX  RotationSequenceAngles=[0 0 0]  RotationSequenceAnglesUnits=deg  RotationMatrix=[1 0 0; 0 1 0; 0 0 1]  Quaternion=[1 0 0 0]  TranslationMethod=Cartesian  TranslationCartesianOffset=[0, 0, 0]  TranslationCartesianOffsetUnits=m  TranslationStandardAxis=+Z  TranslationStandardOffset=0  TranslationStandardOffsetUnits=m  TranslationROffset=0  TranslationROffsetUnits=m  TranslationThetaOffset=0  TranslationThetaOffsetUnits=deg  TranslationZOffset=0  TranslationZOffsetUnits=m
  panda_joint2_AxisTransform : sm_lib/Frames and Transforms/Rigid Transform  RotationMethod=ArbitraryAxis  FollAlignAxisA=+X  BaseAlignAxisA=+Y  FollAlignAxisB=+Y  BaseAlignAxisB=+Z  RotationStandardAxis=+Z  RotationAngle=0  RotationAngleUnits=rad  RotationArbitraryAxis=[1, 0, 0]  RotationSequenceAxes=FollowerAxes  RotationSequence=XYX  RotationSequenceAngles=[0 0 0]  RotationSequenceAnglesUnits=deg  RotationMatrix=[1 0 0; 0 1 0; 0 0 1]  Quaternion=[1 0 0 0]  TranslationMethod=Cartesian  TranslationCartesianOffset=[0, 0, 0]  TranslationCartesianOffsetUnits=m  TranslationStandardAxis=+Z  TranslationStandardOffset=0  TranslationStandardOffsetUnits=m  TranslationROffset=0  TranslationROffsetUnits=m  TranslationThetaOffset=0  TranslationThetaOffsetUnits=deg  TranslationZOffset=0  TranslationZOffsetUnits=m
  panda_joint2_OriginTransform : sm_lib/Frames and Transforms/Rigid Transform  RotationMethod=RotationSequence  FollAlignAxisA=+X  BaseAlignAxisA=+Y  FollAlignAxisB=+Y  BaseAlignAxisB=+Z  RotationStandardAxis=+Z  RotationAngle=0.0  RotationAngleUnits=deg  RotationArbitraryAxis=[0 0 1]  RotationSequenceAxes=BaseAxes  RotationSequence=XYZ  RotationSequenceAngles=[-1.57079632679, 0, 0]  RotationSequenceAnglesUnits=rad  RotationMatrix=[1 0 0; 0 1 0; 0 0 1]  Quaternion=[1 0 0 0]  TranslationMethod=Cartesian  TranslationCartesianOffset=[0, 0, 0]  TranslationCartesianOffsetUnits=m  TranslationStandardAxis=+Z  TranslationStandardOffset=0  TranslationStandardOffsetUnits=m  TranslationROffset=0  TranslationROffsetUnits=m  TranslationThetaOffset=0  TranslationThetaOffsetUnits=deg  TranslationZOffset=0  TranslationZOffsetUnits=m
  F : PMIOPort  Side=Left
  F1 : PMIOPort  Port=2  Side=Right
  connections:
  Inertia/RConn1 -- InertiaOriginTransform/RConn1
  ReferenceFrame/RConn1 -- InertiaOriginTransform/LConn1 -- panda_joint1_AxisInvTransform/LConn1 -- panda_joint2_OriginTransform/LConn1 -- VisualOriginTransform/LConn1
  Visual/RConn1 -- VisualOriginTransform/RConn1
  panda_joint1_AxisInvTransform/RConn1 -- F/RConn1
  panda_joint2_AxisTransform/RConn1 -- F1/RConn1
  panda_joint2_AxisTransform/LConn1 -- panda_joint2_OriginTransform/RConn1

== system Controller_torque_cbf/Franka Forward Dynamics2/Franka Forward Dynamics [SimMechanics]/panda_link2 ==
  Inertia : sm_lib/Body Elements/Inertia  InertiaType=Custom  Mass=0.646926  MassUnits=kg  CenterOfMass=[0, 0, 0]  CenterOfMassUnits=m  MomentsOfInertia=[0.007962, 0.02811, 0.025995]  MomentsOfInertiaUnits=kg*m^2  ProductsOfInertia=[0.000704, 0.010254, -0.003925]  ProductsOfInertiaUnits=kg*m^2  GraphicType=None  MarkerShape=Inertia  MarkerSize=20  GraphicVisPropType=SimpleVisualProperties  GraphicDiffuseColor=[0.5 0.5 0.5]  GraphicOpacity=1.0  GraphicSpecularColor=[0.5 0.5 0.5 1.0]  GraphicAmbientColor=[0.15 0.15 0.15 1.0]  GraphicEmissiveColor=[0.0 0.0 0.0 1.0]  GraphicShininess=75
  InertiaOriginTransform : sm_lib/Frames and Transforms/Rigid Transform  RotationMethod=RotationSequence  FollAlignAxisA=+X  BaseAlignAxisA=+Y  FollAlignAxisB=+Y  BaseAlignAxisB=+Z  RotationStandardAxis=+Z  RotationAngle=0.0  RotationAngleUnits=deg  RotationArbitraryAxis=[0 0 1]  RotationSequenceAxes=BaseAxes  RotationSequence=XYZ  RotationSequenceAngles=[0, 0, 0]  RotationSequenceAnglesUnits=rad  RotationMatrix=[1 0 0; 0 1 0; 0 0 1]  Quaternion=[1 0 0 0]  TranslationMethod=Cartesian  TranslationCartesianOffset=[-0.003141, -0.02872, 0.003495]  TranslationCartesianOffsetUnits=m  TranslationStandardAxis=+Z  TranslationStandardOffset=0  TranslationStandardOffsetUnits=m  TranslationROffset=0  TranslationROffsetUnits=m  TranslationThetaOffset=0  TranslationThetaOffsetUnits=deg  TranslationZOffset=0  TranslationZOffsetUnits=m
  ReferenceFrame : sm_lib/Frames and Transforms/Reference Frame
  Visual : sm_lib/Body Elements/File Solid  ExtGeomFileName=RobotFiles/Franka_Panda/meshes/visual/link2-Mesh.stl  UnitType=Custom  ExtGeomFileUnits=mm  StepReaderType=HEX  ExportConvexHullGeometry=off  InertiaType=Custom  BasedOnType=DensityFromFile  Density=1000  DensityUnits=kg/m^3  Mass=0  MassUnits=kg  CenterOfMass=[0, 0, 0]  CenterOfMassUnits=m  MomentsOfInertia=[0, 0, 0]  MomentsOfInertiaUnits=kg*m^2  ProductsOfInertia=[0, 0, 0]  ProductsOfInertiaUnits=kg*m^2  GraphicType=FromGeometry  MarkerShape=Sphere  MarkerSize=10  GraphicVisPropType=SimpleVisualProperties  GraphicDiffuseColor=[1.0 1.0 1.0]  GraphicOpacity=1  GraphicSpecularColor=[0.5 0.5 0.5 1.0]  GraphicAmbientColor=[0.15 0.15 0.15 1.0]  GraphicEmissiveColor=[0.0 0.0 0.0 1.0]  GraphicShininess=75  DoExposeReferenceFrame=on  SerializedFrames=<Frames/>
  VisualOriginTransform : sm_lib/Frames and Transforms/Rigid Transform  RotationMethod=RotationSequence  FollAlignAxisA=+X  BaseAlignAxisA=+Y  FollAlignAxisB=+Y  BaseAlignAxisB=+Z  RotationStandardAxis=+Z  RotationAngle=0.0  RotationAngleUnits=deg  RotationArbitraryAxis=[0 0 1]  RotationSequenceAxes=BaseAxes  RotationSequence=XYZ  RotationSequenceAngles=[0, 0, 0]  RotationSequenceAnglesUnits=rad  RotationMatrix=[1 0 0; 0 1 0; 0 0 1]  Quaternion=[1 0 0 0]  TranslationMethod=Cartesian  TranslationCartesianOffset=[0, 0, 0]  TranslationCartesianOffsetUnits=m  TranslationStandardAxis=+Z  TranslationStandardOffset=0  TranslationStandardOffsetUnits=m  TranslationROffset=0  TranslationROffsetUnits=m  TranslationThetaOffset=0  TranslationThetaOffsetUnits=deg  TranslationZOffset=0  TranslationZOffsetUnits=m
  panda_joint2_AxisInvTransform : sm_lib/Frames and Transforms/Rigid Transform  RotationMethod=ArbitraryAxis  FollAlignAxisA=+X  BaseAlignAxisA=+Y  FollAlignAxisB=+Y  BaseAlignAxisB=+Z  RotationStandardAxis=+Z  RotationAngle=0  RotationAngleUnits=rad  RotationArbitraryAxis=[1, 0, 0]  RotationSequenceAxes=FollowerAxes  RotationSequence=XYX  RotationSequenceAngles=[0 0 0]  RotationSequenceAnglesUnits=deg  RotationMatrix=[1 0 0; 0 1 0; 0 0 1]  Quaternion=[1 0 0 0]  TranslationMethod=Cartesian  TranslationCartesianOffset=[0, 0, 0]  TranslationCartesianOffsetUnits=m  TranslationStandardAxis=+Z  TranslationStandardOffset=0  TranslationStandardOffsetUnits=m  TranslationROffset=0  TranslationROffsetUnits=m  TranslationThetaOffset=0  TranslationThetaOffsetUnits=deg  TranslationZOffset=0  TranslationZOffsetUnits=m
  panda_joint3_AxisTransform : sm_lib/Frames and Transforms/Rigid Transform  RotationMethod=ArbitraryAxis  FollAlignAxisA=+X  BaseAlignAxisA=+Y  FollAlignAxisB=+Y  BaseAlignAxisB=+Z  RotationStandardAxis=+Z  RotationAngle=0  RotationAngleUnits=rad  RotationArbitraryAxis=[1, 0, 0]  RotationSequenceAxes=FollowerAxes  RotationSequence=XYX  RotationSequenceAngles=[0 0 0]  RotationSequenceAnglesUnits=deg  RotationMatrix=[1 0 0; 0 1 0; 0 0 1]  Quaternion=[1 0 0 0]  TranslationMethod=Cartesian  TranslationCartesianOffset=[0, 0, 0]  TranslationCartesianOffsetUnits=m  TranslationStandardAxis=+Z  TranslationStandardOffset=0  TranslationStandardOffsetUnits=m  TranslationROffset=0  TranslationROffsetUnits=m  TranslationThetaOffset=0  TranslationThetaOffsetUnits=deg  TranslationZOffset=0  TranslationZOffsetUnits=m
  panda_joint3_OriginTransform : sm_lib/Frames and Transforms/Rigid Transform  RotationMethod=RotationSequence  FollAlignAxisA=+X  BaseAlignAxisA=+Y  FollAlignAxisB=+Y  BaseAlignAxisB=+Z  RotationStandardAxis=+Z  RotationAngle=0.0  RotationAngleUnits=deg  RotationArbitraryAxis=[0 0 1]  RotationSequenceAxes=BaseAxes  RotationSequence=XYZ  RotationSequenceAngles=[1.57079632679, 0, 0]  RotationSequenceAnglesUnits=rad  RotationMatrix=[1 0 0; 0 1 0; 0 0 1]  Quaternion=[1 0 0 0]  TranslationMethod=Cartesian  TranslationCartesianOffset=[0, -0.316, 0]  TranslationCartesianOffsetUnits=m  TranslationStandardAxis=+Z  TranslationStandardOffset=0  TranslationStandardOffsetUnits=m  TranslationROffset=0  TranslationROffsetUnits=m  TranslationThetaOffset=0  TranslationThetaOffsetUnits=deg  TranslationZOffset=0  TranslationZOffsetUnits=m
  F : PMIOPort  Side=Left
  F1 : PMIOPort  Port=2  Side=Right
  connections:
  Inertia/RConn1 -- InertiaOriginTransform/RConn1
  ReferenceFrame/RConn1 -- InertiaOriginTransform/LConn1 -- panda_joint2_AxisInvTransform/LConn1 -- panda_joint3_OriginTransform/LConn1 -- VisualOriginTransform/LConn1
  Visual/RConn1 -- VisualOriginTransform/RConn1
  panda_joint2_AxisInvTransform/RConn1 -- F/RConn1
  panda_joint3_AxisTransform/RConn1 -- F1/RConn1
  panda_joint3_AxisTransform/LConn1 -- panda_joint3_OriginTransform/RConn1
